simulink model "pack_topology"  (R2026a)
settings: Solver=VariableStepAuto
libraries: fl_lib x19
settings Model: Creator=yashi  LastModifiedBy=yashi

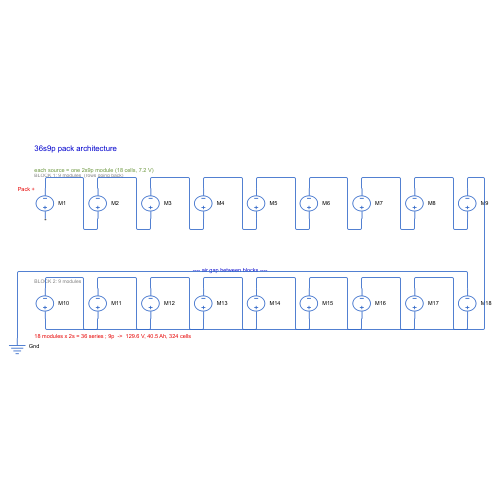
[thumbnail: Simulink's stored preview of the top-level diagram]
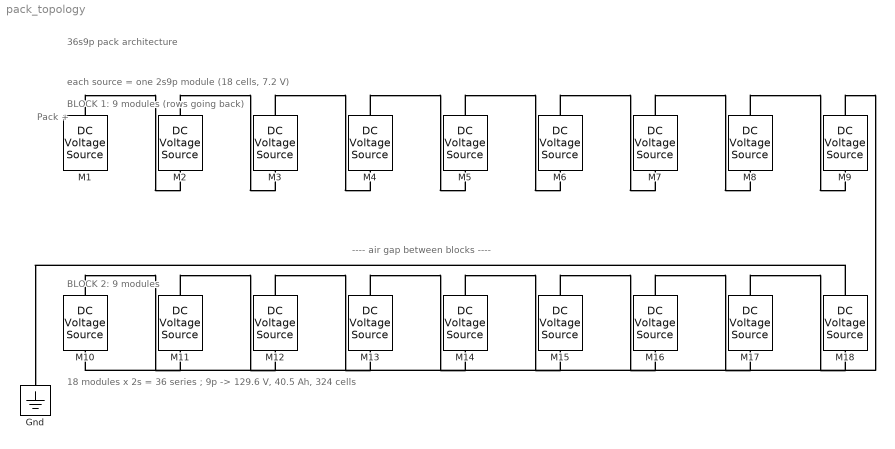
== system pack_topology ==
  note: 36s9p pack architecture
  note: each source = one 2s9p module (18 cells, 7.2 V)
  note: BLOCK 1: 9 modules (rows going back)
  note: ---- air gap between blocks ----
  note: BLOCK 2: 9 modules
  note: 18 modules x 2s = 36 series ; 9p -> 129.6 V, 40.5 Ah, 324 cells
  note: Pack +
  Gnd : fl_lib/Electrical/Electrical Elements/Electrical Reference
  M{1..18} (18 alike) : fl_lib/Electrical/Electrical Sources/DC Voltage Source  v0=7.2 V
  connections:
  M1/RConn1 -- M2/LConn1
  M2/RConn1 -- M3/LConn1
  M3/RConn1 -- M4/LConn1
  M4/RConn1 -- M5/LConn1
  M5/RConn1 -- M6/LConn1
  M6/RConn1 -- M7/LConn1
  M7/RConn1 -- M8/LConn1
  M8/RConn1 -- M9/LConn1
  M9/RConn1 -- M10/LConn1
  M10/RConn1 -- M11/LConn1
  M11/RConn1 -- M12/LConn1
  M12/RConn1 -- M13/LConn1
  M13/RConn1 -- M14/LConn1
  M14/RConn1 -- M15/LConn1
  M15/RConn1 -- M16/LConn1
  M16/RConn1 -- M17/LConn1
  M17/RConn1 -- M18/LConn1
  M18/RConn1 -- Gnd/LConn1
